simulink model "pid_dependen_stick"  (R2025a)
settings: Solver=VariableStepAuto  StartTime=0.0  StopTime=5  RelTol=1e-3
undefined symbols (not defined in the file): Kp, Td, Ti
settings Model: Creator=Acer  LastModifiedBy=Acer

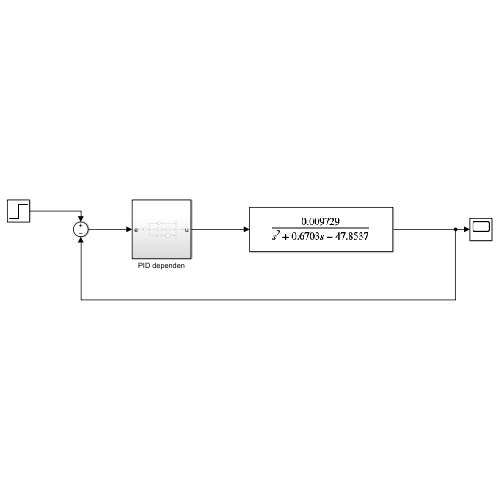
[thumbnail: Simulink's stored preview of the top-level diagram]
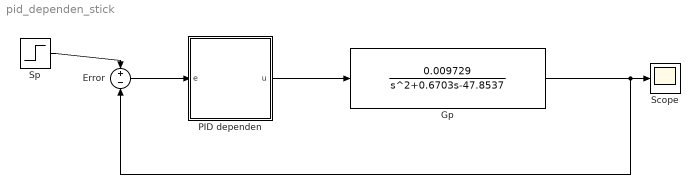
== system pid_dependen_stick ==
  Error : Sum  Inputs=+-
  Gp : TransferFcn  Numerator=0.009729  Denominator=[1 0.6703 -47.8537]
  PID dependen : Subsystem
  Scope : Scope
      settings: ActiveDisplayYMinimum=-0.051916413297269211  ActiveDisplayYMaximum=0.467247719675423
  Sp : Step  Time=0  After=0.087  SampleTime=0
  wires:
  Sp/1 -> Error/1
  Error/1 -> PID dependen/1(e)
  PID dependen/1(u) -> Gp/1
  Gp/1 -> Scope/1, Error/2

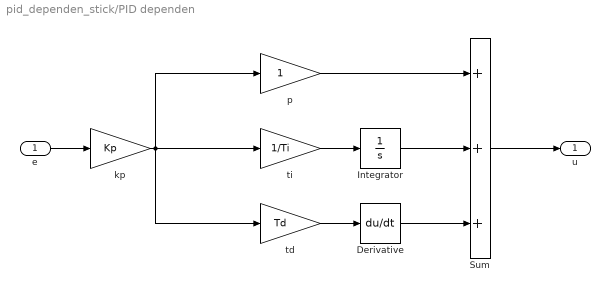
== system pid_dependen_stick/PID dependen ==
  e : Inport
  Derivative : Derivative
  Integrator : Integrator
  Sum : Sum  Inputs=+++
  kp : Gain  Gain=Kp
  p : Gain
  td : Gain  Gain=Td
  ti : Gain  Gain=1/Ti
  u : Outport
  wires:
  e/1 -> kp/1
  p/1 -> Sum/1
  ti/1 -> Integrator/1
  Integrator/1 -> Sum/2
  td/1 -> Derivative/1
  Derivative/1 -> Sum/3
  Sum/1 -> u/1
  kp/1 -> p/1, td/1, ti/1
